simulink model "inv_im_param"  (R2026b)
settings: Solver=ode23tb  StopTime=param.sim.simlength  FixedStep=tc  MaxStep=param.glb_time.tc
values from neighbouring files (symbols this model uses):
  param = add_template_extras(param, options)    [init_model.m]
undefined symbols (not defined in the file or in its folder): magnitude
libraries: fl_lib x30, nesl_utility x13, lithium_ion_battery x1, induction_machine x1, dclink_with_center_tap x1, dead_time_generator_cmos_simulink x1, three_phase_pwm_modulator x1, three_phase_inverter_ideal_switch_based_model x1, three_phase_inverter_igbt_advanced_thermal_model x1, three_phase_inverter_mosfet_based_with_thermal_model x1, threephase_inductor_lib x1, simple_flexible_shaft x1
(part 1 of 3)
settings Model: Creator=dbagn  LastModifiedBy=d.bagnara
settings SolverCC: SolverResetMethod=Robust  ZeroCrossControl=DisableAll
settings DataIOCC: DSMLogging=off  ReturnWorkspaceOutputs=off  SaveOutput=off  SaveTime=off  SignalLogging=off
settings OptimizationCC: ReuseModelBlockBuffer=off
settings SFSimCC: CustomCodeUndefinedFunction=ThrowError  DefaultCustomCodeDeterministicFunctions=All
settings SFSimCC: SimCustomHeaderCode=|
  | #include "rpi.h"
  | #include "mavgflt.h"
  | #include "mavgflt_simulink.h"
  | #include "mavgflts.h"
  | #include "mavgflts_simulink.h"
  | #include "dsmavgflt.h"
  | #include "dsmavgflt_simulink.h"
  | #include "bemf_obsv.h"
  | #include "bemf_obsv_simulink.h"
  | #include "bemf_obsv_load_est.h"
  | #include "bemf_obsv_load_est_simulink.h"
  | #include "dqvector_pi.h"
  | #include "dqvector_pi_simulink.h"
  | #include "sv_pwm_simulink.h"
  | #include "sv_pwm.h"
  | #include "first_harmonic_tracker.h"
  | #include "first_harmonic_tracker_simulink.h"
  | #include "dqpll_thyr.h"
  | #include "dqpll_thyr_simulink.h"
  | #include "dqpll_grid.h"
  | #include "dqpll_grid_simulink.h"
settings SFSimCC: SimUserIncludeDirs=|
  | include
  | src
settings SFSimCC: SimUserSources=|
  | "rpi.c"
  | "mavgflt_simulink.c"
  | "mavgflt.c"
  | "mavgflts_simulink.c"
  | "mavgflts.c"
  | "dsmavgflt_simulink.c"
  | "dsmavgflt.c"
  | "bemf_obsv_simulink.c"
  | "bemf_obsv.c"
  | "bemf_obsv_load_est_simulink.c"
  | "bemf_obsv_load_est.c"
  | "dqvector_pi.c"
  | "dqvector_pi_simulink.c"
  | "sv_pwm_simulink.c"
  | "sv_pwm.c"
  | "first_harmonic_tracker_simulink.c"
  | "first_harmonic_tracker.c"
  | "dqpll_thyr_simulink.c"
  | "dqpll_thyr.c"
  | "dqpll_grid_simulink.c"
  | "dqpll_grid.c"
settings RTWCC: DLArmComputeVersion=19.05
settings SimscapeCC: SimscapeUseEnergyAccounting=off

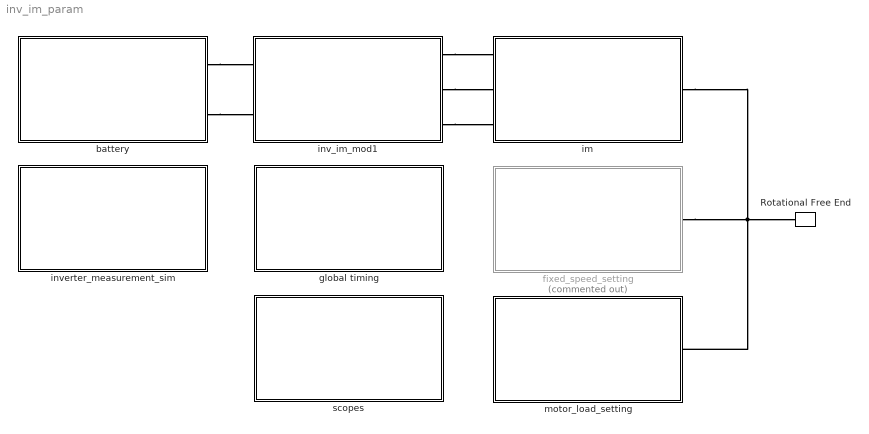
== system inv_im_param ==
  Rotational Free End : fl_lib/Mechanical/Rotational Elements/Rotational Free End  w_specify=off  w_priority=None  w=0 rad/s  w_nominal_specify=off  w_nominal_value=1  w_nominal_unit=rad/s
  battery : Subsystem
  fixed_speed_setting : Subsystem  Commented=on
  global timing : Subsystem
  im : Subsystem
  inv_im_mod1 : Subsystem
  inverter_measurement_sim : Subsystem
  motor_load_setting : Subsystem
  scopes : Subsystem
  connections:
  im/RConn1 -- motor_load_setting/LConn1 -- Rotational Free End/LConn1 -- fixed_speed_setting/LConn1
  inv_im_mod1/RConn2 -- im/LConn2
  inv_im_mod1/RConn1 -- im/LConn1
  inv_im_mod1/RConn3 -- im/LConn3
  battery/RConn1 -- inv_im_mod1/LConn1
  battery/RConn2 -- inv_im_mod1/LConn2

== system inv_im_param/battery ==
  Solver Configuration : nesl_utility/Solver Configuration  PhysicalDomain=network_engine_domain  SubClassName=solver  LeftPortType=input  RightPortType=generic  Tones=[]  Harmonics=[]  SimulateNoise=off  Profile=off  UseLocalSampling=off  EnableSwitchedLinearOptims=on  FrequencyDomain=off  UseCCode=off  RelTol=0.001  AbsTol=0.001  MinStep=1e-09  ToWorkspace=off  RevertToSquareIcSolve=off  NumHomotopyIterations=100  PhasorMode=off  PhasorModeNumHarmonics=1  ConsistencySolver=NEWTON_FTOL  CanonicalOrdering=UNORDERED  OptimizeIntermediates=UNOPTIMIZED  MulticoreSolverChoice=BACKWARD_EULER  IndexReductionMethod=DerivativeReplacement  DoDC=on  ResidualTolerance=1e-3  ConsistencyTolSource=GLOBAL  ConsistencyAbsTol=0.001  ConsistencyRelTol=0.001  ConsistencyTolFactor=0.001  UseLocalSolver=on  LocalSolverChoice=NE_BACKWARD_EULER_ADVANCER  ResolveIndetEquations=on  FunctionEvalNumThread=1  LocalSolverSampleTime=param.glb_time.tc  DoFixedCost=on  MaxNonlinIter=param.sim.nonlinear_iterations  MaxModeIter=2  ComputeImpulses=off  ImpulseIterations=2  LinearAlgebra=auto  LinearAlgebraNumThread=0  EquationFormulation=NE_TIME_EF  DelaysMemoryBudget=1024  AutomaticFiltering=on  FilteringTimeConstant=0.001  PartitionStorageMethod=AS_NEEDED  PartitionMemoryBudget=1024  PartitionMethod=BALANCED  MultibodyUseLocalSolver=off  MultibodyLocalSolverChoice=ODE1  MultibodyLocalSolverSampleTime=0.001
  To Workspace14 : ToWorkspace  VariableName=battery_data  SampleTime=param.glb_time.tc
      settings: MaxDataPoints=param.glb_time.Nc  Decimation=param.glb_time.decimation_tc
  lithium-ion_battery : lithium_ion_battery/lithium_ion_battery  Q=param.battery.pack_1.Q  number_of_cells=param.battery.pack_1.number_of_cells  E_1=param.battery.pack_1.E_1  E0=param.battery.pack_1.E0  E1=param.battery.pack_1.E1  E2=param.battery.pack_1.E2  E3=param.battery.pack_1.E3  Elog=param.battery.pack_1.Elog  R0=param.battery.pack_1.R0  R1=param.battery.pack_1.R1  C1=param.battery.pack_1.C1  M=param.battery.pack_1.M  alpha=param.battery.pack_1.alpha  soc_init=param.battery.pack_1.soc_init  ts_battery=param.glb_time.ts_dab  q1Kalman=param.battery.pack_1.q1Kalman  q2Kalman=param.battery.pack_1.q2Kalman  q3Kalman=param.battery.pack_1.q3Kalman  rKalman=param.battery.pack_1.rKalman  tc=param.glb_time.tc  enable_white_noise_m=0  battery_voltage_init_m=param.battery.nominal_battery_voltage_1
  litium ion battery : Scope
      settings: ActiveDisplayYMinimum=-388.27149612119968  ActiveDisplayYMaximum=1221.0011073633038  DataLoggingVariableName=ScopeData3
  single_phase_ui_measure : Subsystem
  dc+ : PMIOPort  Side=Right
  dc- : PMIOPort  Port=2  Side=Right
  wires:
  lithium-ion_battery/1 -> To Workspace14/1, litium ion battery/1
  connections:
  single_phase_ui_measure/LConn2 -- lithium-ion_battery/RConn2 -- Solver Configuration/RConn1
  single_phase_ui_measure/RConn1 -- dc+/RConn1
  lithium-ion_battery/RConn1 -- single_phase_ui_measure/LConn1
  dc-/RConn1 -- single_phase_ui_measure/RConn2

== system inv_im_param/fixed_speed_setting ==
  Ideal Angular Velocity Source : fl_lib/Mechanical/Mechanical Sources/Ideal Angular Velocity Source
  Mechanical Rotational Reference : fl_lib/Mechanical/Rotational Elements/Mechanical Rotational Reference
  PS Step1 : fl_lib/Physical Signals/Sources/PS Step  step_time=0.025 s  initial_value=0 rpm  final_value=param.load.rpm_sim rpm
  PS Transfer Function : fl_lib/Physical Signals/Linear Operators/PS Transfer Function  transfer_function_type=foundation.enum.transfer_function_type.lag  T=0.1 s  T1=2 s  T2=1 s  reset_method=foundation.enum.IntegratorResetSpec.None  initial_condition_spec=foundation.enum.IntegratorICSpec.Internal  y0=0 rpm
  shaft : PMIOPort  Side=Left
  connections:
  Mechanical Rotational Reference/LConn1 -- Ideal Angular Velocity Source/RConn2
  PS Step1/RConn1 -- PS Transfer Function/LConn1
  PS Transfer Function/RConn1 -- Ideal Angular Velocity Source/RConn1
  Ideal Angular Velocity Source/LConn1 -- shaft/RConn1

== system inv_im_param/global timing ==
  Unit Delay : UnitDelay  SampleTime=param.glb_time.tc
  Unit Delay1 : UnitDelay  SampleTime=param.glb_time.tc
  time_afe1 : Subsystem  mask{k=param.afe.behav.time_gain_module_1}
      mask prompts: k "Time Gain"
      mask Display:
      | disp('time-gen');
      | port_label('input', 1, 'crt');
      | port_label('output', 1, 'tout');
  time_afe3 : Subsystem  mask{k=1}
      mask prompts: k "Time Gain"
      mask Display:
      | disp('time-gen');
      | port_label('output', 1, 'tout');
  time_inv1 : Subsystem  mask{k=param.inv.behav.time_gain_module_2}
      mask prompts: k "Time Gain"
      mask Display:
      | disp('time-gen');
      | port_label('input', 1, 'crt');
      | port_label('output', 1, 'tout');
  tag scope: time_afe_module_1=global, time_inv_module_1=global, time_master=global
  wires:
  time_afe1/1(Out1) -> [time_afe_module_1]
  time_inv1/1(Out1) -> [time_inv_module_1]
  time_afe3/1(Out1) -> [time_master]
  [local_time_corr_afe1] -> Unit Delay/1
  Unit Delay/1 -> time_afe1/1(correction_time)
  [local_time_corr_inv1] -> Unit Delay1/1
  Unit Delay1/1 -> time_inv1/1(correction_time)

== system inv_im_param/im ==
  Bus Selector1 : BusSelector  OutputSignals=rotor_speed_electrical(rad/s)
  im_machine : Subsystem
  u : PMIOPort  Side=Left
  v : PMIOPort  Port=2  Side=Left
  w : PMIOPort  Port=3  Side=Left
  shaft : PMIOPort  Port=4  Side=Right
  tag scope: rotor_speed_electrical_im=global
  wires:
  im_machine/1(motor_data) -> Bus Selector1/1
  Bus Selector1/1 -> [rotor_speed_electrical_im]  "<rotor_speed_electrical(rad/s)>"
  connections:
  im_machine/LConn1 -- u/RConn1
  im_machine/LConn3 -- w/RConn1
  im_machine/LConn2 -- v/RConn1
  shaft/RConn1 -- im_machine/RConn1

== system inv_im_param/inv_im_mod1 ==
  dc_source : Subsystem
  inverter : Subsystem
  inverter_ctrl : Subsystem
  output_filter : Subsystem
  us_u : PMIOPort  Side=Right
  us_v : PMIOPort  Port=2  Side=Right
  us_w : PMIOPort  Port=3  Side=Right
  udc(+) : PMIOPort  Port=4  Side=Left
  udc(-) : PMIOPort  Port=5  Side=Left
  wires:
  inverter_ctrl/1(duvw_out) -> inverter/1(duvw)
  connections:
  inverter/LConn2 -- output_filter/RConn2
  inverter/LConn1 -- output_filter/RConn1
  inverter/LConn3 -- output_filter/RConn3
  output_filter/LConn2 -- us_v/RConn1
  output_filter/LConn3 -- us_w/RConn1
  output_filter/LConn1 -- us_u/RConn1
  dc_source/RConn1 -- inverter/RConn1
  inverter/RConn2 -- dc_source/RConn2
  dc_source/LConn2 -- udc(-)/RConn1
  dc_source/LConn1 -- udc(+)/RConn1

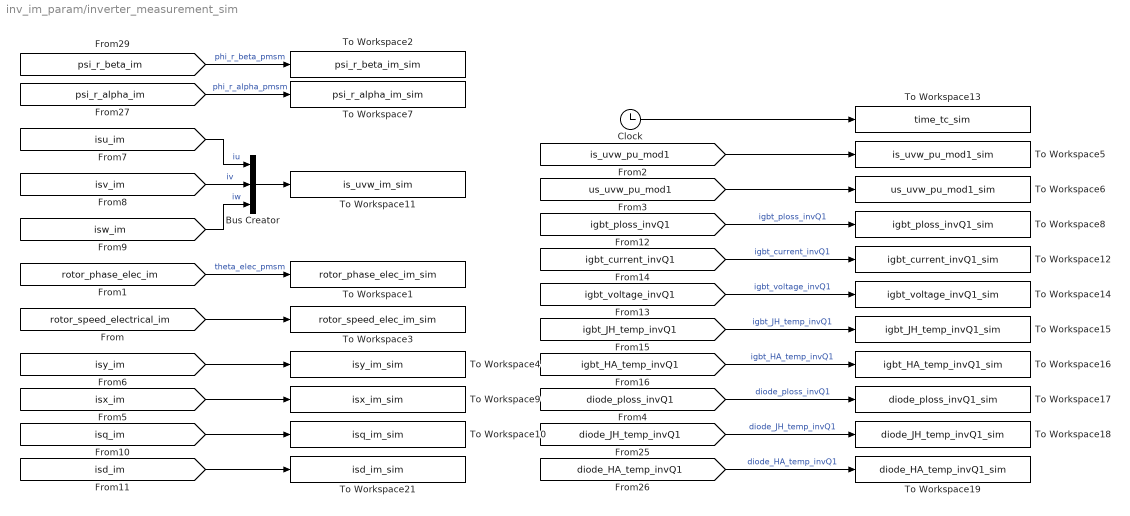
== system inv_im_param/inverter_measurement_sim ==
  Bus Creator : BusCreator  Inputs=3
  Clock : Clock
  To Workspace1 : ToWorkspace  VariableName=rotor_phase_elec_im_sim  SampleTime=param.glb_time.tc
      settings: MaxDataPoints=param.glb_time.Nc  Decimation=param.glb_time.decimation_tc
  To Workspace10 : ToWorkspace  VariableName=isq_im_sim  SampleTime=param.glb_time.tc
      settings: MaxDataPoints=param.glb_time.Nc  Decimation=param.glb_time.decimation_tc
  To Workspace11 : ToWorkspace  VariableName=is_uvw_im_sim  SampleTime=param.glb_time.tc
      settings: MaxDataPoints=param.glb_time.Nc  Decimation=param.glb_time.decimation_tc
  To Workspace12 : ToWorkspace  VariableName=igbt_current_invQ1_sim  SampleTime=param.glb_time.tc
      settings: MaxDataPoints=param.glb_time.Nc  Decimation=param.glb_time.decimation_tc
  To Workspace13 : ToWorkspace  VariableName=time_tc_sim  SampleTime=param.glb_time.tc
      settings: MaxDataPoints=param.glb_time.Nc  Decimation=param.glb_time.decimation_tc
  To Workspace14 : ToWorkspace  VariableName=igbt_voltage_invQ1_sim  SampleTime=param.glb_time.tc
      settings: MaxDataPoints=param.glb_time.Nc  Decimation=param.glb_time.decimation_tc
  To Workspace15 : ToWorkspace  VariableName=igbt_JH_temp_invQ1_sim  SampleTime=param.glb_time.tc
      settings: MaxDataPoints=param.glb_time.Nc  Decimation=param.glb_time.decimation_tc
  To Workspace16 : ToWorkspace  VariableName=igbt_HA_temp_invQ1_sim  SampleTime=param.glb_time.tc
      settings: MaxDataPoints=param.glb_time.Nc  Decimation=param.glb_time.decimation_tc
  To Workspace17 : ToWorkspace  VariableName=diode_ploss_invQ1_sim  SampleTime=param.glb_time.tc
      settings: MaxDataPoints=param.glb_time.Nc  Decimation=param.glb_time.decimation_tc
  To Workspace18 : ToWorkspace  VariableName=diode_JH_temp_invQ1_sim  SampleTime=param.glb_time.tc
      settings: MaxDataPoints=param.glb_time.Nc  Decimation=param.glb_time.decimation_tc
  To Workspace19 : ToWorkspace  VariableName=diode_HA_temp_invQ1_sim  SampleTime=param.glb_time.tc
      settings: MaxDataPoints=param.glb_time.Nc  Decimation=param.glb_time.decimation_tc
  To Workspace2 : ToWorkspace  VariableName=psi_r_beta_im_sim  SampleTime=param.glb_time.tc
      settings: MaxDataPoints=param.glb_time.Nc  Decimation=param.glb_time.decimation_tc
  To Workspace21 : ToWorkspace  VariableName=isd_im_sim  SampleTime=param.glb_time.tc
      settings: MaxDataPoints=param.glb_time.Nc  Decimation=param.glb_time.decimation_tc
  To Workspace3 : ToWorkspace  VariableName=rotor_speed_elec_im_sim  SampleTime=param.glb_time.tc
      settings: MaxDataPoints=param.glb_time.Nc  Decimation=param.glb_time.decimation_tc
  To Workspace4 : ToWorkspace  VariableName=isy_im_sim  SampleTime=param.glb_time.tc
      settings: MaxDataPoints=param.glb_time.Nc  Decimation=param.glb_time.decimation_tc
  To Workspace5 : ToWorkspace  VariableName=is_uvw_pu_mod1_sim  SampleTime=param.glb_time.tc
      settings: MaxDataPoints=param.glb_time.Nc  Decimation=param.glb_time.decimation_tc
  To Workspace6 : ToWorkspace  VariableName=us_uvw_pu_mod1_sim  SampleTime=param.glb_time.tc
      settings: MaxDataPoints=param.glb_time.Nc  Decimation=param.glb_time.decimation_tc
  To Workspace7 : ToWorkspace  VariableName=psi_r_alpha_im_sim  SampleTime=param.glb_time.tc
      settings: MaxDataPoints=param.glb_time.Nc  Decimation=param.glb_time.decimation_tc
  To Workspace8 : ToWorkspace  VariableName=igbt_ploss_invQ1_sim  SampleTime=param.glb_time.tc
      settings: MaxDataPoints=param.glb_time.Nc  Decimation=param.glb_time.decimation_tc
  To Workspace9 : ToWorkspace  VariableName=isx_im_sim  SampleTime=param.glb_time.tc
      settings: MaxDataPoints=param.glb_time.Nc  Decimation=param.glb_time.decimation_tc
  wires:
  [psi_r_alpha_im] -> To Workspace7/1  "phi_r_alpha_pmsm"
  [psi_r_beta_im] -> To Workspace2/1  "phi_r_beta_pmsm"
  [rotor_speed_electrical_im] -> To Workspace3/1
  [isv_im] -> Bus Creator/2  "iv"
  [isw_im] -> Bus Creator/3  "iw"
  [isu_im] -> Bus Creator/1  "iu"
  Bus Creator/1 -> To Workspace11/1
  [rotor_phase_elec_im] -> To Workspace1/1  "theta_elec_pmsm"
  [isy_im] -> To Workspace4/1
  [is_uvw_pu_mod1] -> To Workspace5/1
  [us_uvw_pu_mod1] -> To Workspace6/1
  [igbt_ploss_invQ1] -> To Workspace8/1  "igbt_ploss_invQ1"
  [igbt_current_invQ1] -> To Workspace12/1  "igbt_current_invQ1"
  [igbt_voltage_invQ1] -> To Workspace14/1  "igbt_voltage_invQ1"
  [igbt_JH_temp_invQ1] -> To Workspace15/1  "igbt_JH_temp_invQ1"
  [igbt_HA_temp_invQ1] -> To Workspace16/1  "igbt_HA_temp_invQ1"
  Clock/1 -> To Workspace13/1
  [diode_ploss_invQ1] -> To Workspace17/1  "diode_ploss_invQ1"
  [diode_JH_temp_invQ1] -> To Workspace18/1  "diode_JH_temp_invQ1"
  [diode_HA_temp_invQ1] -> To Workspace19/1  "diode_HA_temp_invQ1"
  [isx_im] -> To Workspace9/1
  [isq_im] -> To Workspace10/1
  [isd_im] -> To Workspace21/1

== system inv_im_param/motor_load_setting ==
  Gain : Gain  Gain=param.im.machine.pp
  Ideal Rotational Motion Sensor : fl_lib/Mechanical/Mechanical Sensors/Ideal Rotational Motion Sensor  reference=foundation.enum.MeasurementReference.difference  acceleration_port=false  velocity_port=true  position_port=true  wrap_angle=false  offset=0 rad
  Ideal Torque Source : fl_lib/Mechanical/Mechanical Sources/Ideal Torque Source
  Inertia : fl_lib/Mechanical/Rotational Elements/Inertia  inertia=param.load.external_load_inertia kg*m^2  num_ports=foundation.enum.numPorts2.one  w_specify=off  w_priority=High  w=0 rad/s  w_nominal_specify=off  w_nominal_value=1  w_nominal_unit=rad/s  t_specify=off  t_priority=None  t=0 N*m  t_nominal_specify=off  t_nominal_value=1  t_nominal_unit=N*m
  Integrator : Integrator
  Mechanical Rotational Reference : fl_lib/Mechanical/Rotational Elements/Mechanical Rotational Reference
  Mechanical Rotational Reference1 : fl_lib/Mechanical/Rotational Elements/Mechanical Rotational Reference
  PS Step : fl_lib/Physical Signals/Sources/PS Step  step_time=param.sim.load_step_time s  initial_value=1 N*m  final_value=1 N*m
  PS Transfer Function : fl_lib/Physical Signals/Linear Operators/PS Transfer Function  transfer_function_type=foundation.enum.transfer_function_type.lag  T=1 s  T1=2 s  T2=1 s  reset_method=foundation.enum.IntegratorResetSpec.None  initial_condition_spec=foundation.enum.IntegratorICSpec.Internal  y0=0 N*m
  PS-Simulink Converter : nesl_utility/PS-Simulink Converter  PhysicalDomain=network_engine_domain  SubClassName=ps_output  LeftPortType=input  RightPortType=output  PseudoPeriodic=off  Frequencies=[]  VectorFormat=1-D array  Unit=rad/s  AffineConversion=off
  PS-Simulink Converter1 : nesl_utility/PS-Simulink Converter  PhysicalDomain=network_engine_domain  SubClassName=ps_output  LeftPortType=input  RightPortType=output  PseudoPeriodic=off  Frequencies=[]  VectorFormat=1-D array  Unit=rpm  AffineConversion=off
  bounder1 : MATLAB Function  TreatAsAtomicUnit=on
  flexible_shaft : simple_flexible_shaft/flexible_shaft  b1=1  b2=1  J1=1  J2=1  b_displacement=1  k_displacement=1e5
  shaft : PMIOPort  Side=Left
  tag scope: encoder_electrical_phase=global, encoder_mechanical_speed=global
  wires:
  PS-Simulink Converter/1 -> Integrator/1
  Integrator/1 -> Gain/1
  Gain/1 -> bounder1/1(u)
  bounder1/1(y) -> [encoder_electrical_phase]
  PS-Simulink Converter1/1 -> [encoder_mechanical_speed]
  connections:
  Ideal Torque Source/LConn1 -- flexible_shaft/RConn1 -- Inertia/LConn1
  Ideal Torque Source/RConn2 -- Mechanical Rotational Reference/LConn1
  PS Transfer Function/RConn1 -- Ideal Torque Source/RConn1
  PS Step/RConn1 -- PS Transfer Function/LConn1
  flexible_shaft/LConn1 -- Ideal Rotational Motion Sensor/LConn1 -- shaft/RConn1
  Ideal Rotational Motion Sensor/RConn1 -- Mechanical Rotational Reference1/LConn1
  Ideal Rotational Motion Sensor/RConn2 -- PS-Simulink Converter1/LConn1 -- PS-Simulink Converter/LConn1

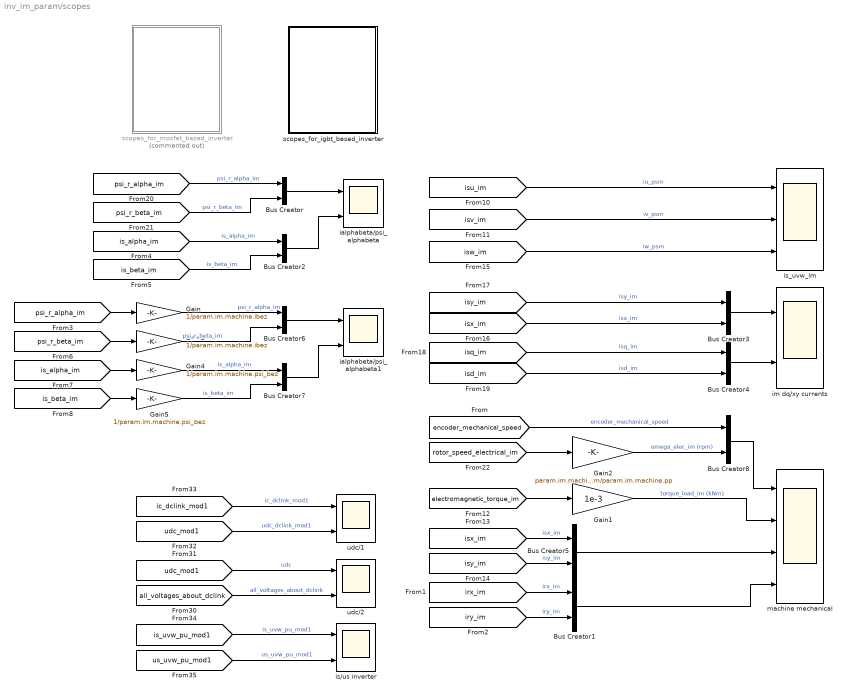
== system inv_im_param/scopes ==
  Bus Creator{,1..8} (9 alike) : BusCreator  Inputs=2
  Gain : Gain  Gain=1/param.im.machine.ibez
  Gain1 : Gain  Gain=1e-3
  Gain2 : Gain  Gain=param.im.machine.radpersecond2rpm/param.im.machine.pp
  Gain3 : Gain  Gain=1/param.im.machine.ibez
  Gain4 : Gain  Gain=1/param.im.machine.psi_bez
  Gain5 : Gain  Gain=1/param.im.machine.psi_bez
  ialphabeta/psi_alphabeta : Scope  NumInputPorts=2
      settings: SampleTime=param.glb_time.tc  ActiveDisplayYMinimum=-1.0786375199515998  ActiveDisplayYMaximum=1.0792953062694595  DataLoggingVariableName=ScopeData17
  ialphabeta/psi_alphabeta1 : Scope  NumInputPorts=2
      settings: SampleTime=param.glb_time.tc  ActiveDisplayYMinimum=-0.0018950393058757126  ActiveDisplayYMaximum=0.0018950920695159389  DataLoggingVariableName=ScopeData18
  im dq/xy currents : Scope  NumInputPorts=2
      settings: SampleTime=param.glb_time.tc  ActiveDisplayYMinimum=-1124.598311193791  ActiveDisplayYMaximum=1120.8872426827804  DataLoggingVariableName=ScopeData7
  is/us inverter : Scope  NumInputPorts=2
      settings: SampleTime=param.glb_time.tc  ActiveDisplayYMinimum=-1.8432109473411751  ActiveDisplayYMaximum=1.8312065303529172  DataLoggingVariableName=ScopeData11
  is_uvw_im : Scope  NumInputPorts=3
      settings: SampleTime=param.glb_time.tc  ActiveDisplayYMinimum=-1113.2920195668116  ActiveDisplayYMaximum=1113.31346416063  DataLoggingVariableName=ScopeData5
  machine mechanical : Scope  NumInputPorts=4
      settings: SampleTime=param.glb_time.tc  ActiveDisplayYMinimum=-18.632200322247279  ActiveDisplayYMaximum=2.78192242658902  DataLoggingVariableName=ScopeData6
  scopes_for_igbt_based_inverter : Subsystem
  scopes_for_mosfet_based_inverter : Subsystem  Commented=on
  udc/1 : Scope  NumInputPorts=2
      settings: SampleTime=param.glb_time.tc  ActiveDisplayYMinimum=-3641.314854214902  ActiveDisplayYMaximum=-3631.7131714883158  DataLoggingVariableName=ScopeData8
  udc/2 : Scope  NumInputPorts=2
      settings: SampleTime=param.glb_time.tc  ActiveDisplayYMinimum=628.98606143046629  ActiveDisplayYMaximum=672.06971446845785  DataLoggingVariableName=ScopeData9
  wires:
  [electromagnetic_torque_im] -> Gain1/1
  Bus Creator4/1 -> im dq/xy currents/2
  [isx_im] -> Bus Creator5/1  "isx_im"
  [isy_im] -> Bus Creator5/2  "isy_im"
  [isw_im] -> is_uvw_im/3  "iw_psm"
  [isd_im] -> Bus Creator4/2  "isd_im"
  [isv_im] -> is_uvw_im/2  "iv_psm"
  Bus Creator3/1 -> im dq/xy currents/1
  [isx_im] -> Bus Creator3/2  "isx_im"
  [isu_im] -> is_uvw_im/1  "iu_psm"
  [isy_im] -> Bus Creator3/1  "isy_im"
  [isq_im] -> Bus Creator4/1  "isq_im"
  [rotor_speed_electrical_im] -> Gain2/1
  [udc_mod1] -> udc/2/1  "udc"
  [ic_dclink_mod1] -> udc/1/1  "ic_dclink_mod1"
  [udc_mod1] -> udc/1/2  "udc_dclink_mod1"
  [all_voltages_about_dclink] -> udc/2/2  "all_voltages_about_dclink"
  [is_uvw_pu_mod1] -> is/us inverter/1  "is_uvw_pu_mod1"
  [us_uvw_pu_mod1] -> is/us inverter/2  "us_uvw_pu_mod1"
  [iry_im] -> Bus Creator1/2  "iry_im"
  [irx_im] -> Bus Creator1/1  "irx_im"
  [psi_r_alpha_im] -> Bus Creator/1  "psi_r_alpha_im"
  [psi_r_beta_im] -> Bus Creator/2  "psi_r_beta_im"
  [is_alpha_im] -> Bus Creator2/1  "is_alpha_im"
  [is_beta_im] -> Bus Creator2/2  "is_beta_im"
  Bus Creator/1 -> ialphabeta/psi_alphabeta/1
  Bus Creator2/1 -> ialphabeta/psi_alphabeta/2
  Bus Creator7/1 -> ialphabeta/psi_alphabeta1/2
  Bus Creator6/1 -> ialphabeta/psi_alphabeta1/1
  [is_beta_im] -> Gain5/1
  [is_alpha_im] -> Gain4/1
  [psi_r_beta_im] -> Gain3/1
  [psi_r_alpha_im] -> Gain/1
  Gain/1 -> Bus Creator6/1  "psi_r_alpha_im"
  Gain3/1 -> Bus Creator6/2  "psi_r_beta_im"
  Gain4/1 -> Bus Creator7/1  "is_alpha_im"
  Gain5/1 -> Bus Creator7/2  "is_beta_im"
  Gain2/1 -> Bus Creator8/2  "omega_elec_im (rpm)"
  [encoder_mechanical_speed] -> Bus Creator8/1  "encoder_mechanical_speed"
  Bus Creator8/1 -> machine mechanical/1
  Gain1/1 -> machine mechanical/2  "torque_load_im (kNm)"
  Bus Creator5/1 -> machine mechanical/3
  Bus Creator1/1 -> machine mechanical/4

== system inv_im_param/battery/single_phase_ui_measure ==
  Bus Creator : BusCreator  Inputs=2
  Current Sensor : fl_lib/Electrical/Electrical Sensors/Current Sensor
  Selector : Selector  InputPortWidth=2  IndexOptions=Index vector (dialog)  Indices=2  OutputSizes=1  RuntimeRangeChecks=off
  Selector1 : Selector  InputPortWidth=2  IndexOptions=Index vector (dialog)  Indices=1  OutputSizes=1  RuntimeRangeChecks=off
  Voltage Sensor : fl_lib/Electrical/Electrical Sensors/Voltage Sensor
  dab input modA : Scope  NumInputPorts=2
      settings: SampleTime=param.glb_time.tc  ActiveDisplayYMinimum=-413.54291450338707  ActiveDisplayYMaximum=396.93489435257015  DataLoggingVariableName=ScopeData2
  iph : nesl_utility/PS-Simulink Converter  PhysicalDomain=network_engine_domain  SubClassName=ps_output  LeftPortType=input  RightPortType=output  PseudoPeriodic=off  Frequencies=[]  VectorFormat=1-D array  Unit=A  AffineConversion=off
  uph : nesl_utility/PS-Simulink Converter  PhysicalDomain=network_engine_domain  SubClassName=ps_output  LeftPortType=input  RightPortType=output  PseudoPeriodic=off  Frequencies=[]  VectorFormat=1-D array  Unit=V  AffineConversion=off
  Udc(+) : PMIOPort  Side=Left
  udc(+) : PMIOPort  Port=2  Side=Right
  Udc(-) : PMIOPort  Port=3  Side=Left
  udc(-) : PMIOPort  Port=4  Side=Right
  tag scope: current_battery=global, voltage_battery=global
  wires:
  Bus Creator/1 -> Selector/1, Selector1/1  "ui_data"
  iph/1 -> Bus Creator/1  "iph"
  uph/1 -> Bus Creator/2  "uph"
  Selector1/1 -> [current_battery], dab input modA/1  "current_battery"
  Selector/1 -> dab input modA/2, [voltage_battery]  "voltage_battery"
  connections:
  iph/LConn1 -- Current Sensor/RConn1
  Voltage Sensor/LConn1 -- Current Sensor/LConn1 -- Udc(+)/RConn1
  Current Sensor/RConn2 -- udc(+)/RConn1
  Voltage Sensor/RConn1 -- uph/LConn1
  Voltage Sensor/RConn2 -- Udc(-)/RConn1 -- udc(-)/RConn1

== system inv_im_param/global timing/time_afe1 ==
  correction_time : Inport
  Constant : Constant
  Gain : Gain  Gain=k
  Product : Product
  Sum : Sum  Inputs=|++
  time_1 : Clock
  Out1 : Outport
  wires:
  time_1/1 -> Gain/1
  Gain/1 -> Product/1
  Product/1 -> Out1/1
  correction_time/1 -> Sum/1
  Sum/1 -> Product/2
  Constant/1 -> Sum/2

== system inv_im_param/global timing/time_afe3 ==
  Gain : Gain  Gain=k
  time_1 : Clock
  Out1 : Outport
  wires:
  Gain/1 -> Out1/1
  time_1/1 -> Gain/1

== system inv_im_param/global timing/time_inv1 ==
  correction_time : Inport
  Constant : Constant
  Gain : Gain  Gain=k
  Product : Product
  Sum : Sum  Inputs=|++
  time_1 : Clock
  Out1 : Outport
  wires:
  time_1/1 -> Gain/1
  Gain/1 -> Product/1
  Product/1 -> Out1/1
  correction_time/1 -> Sum/1
  Constant/1 -> Sum/2
  Sum/1 -> Product/2

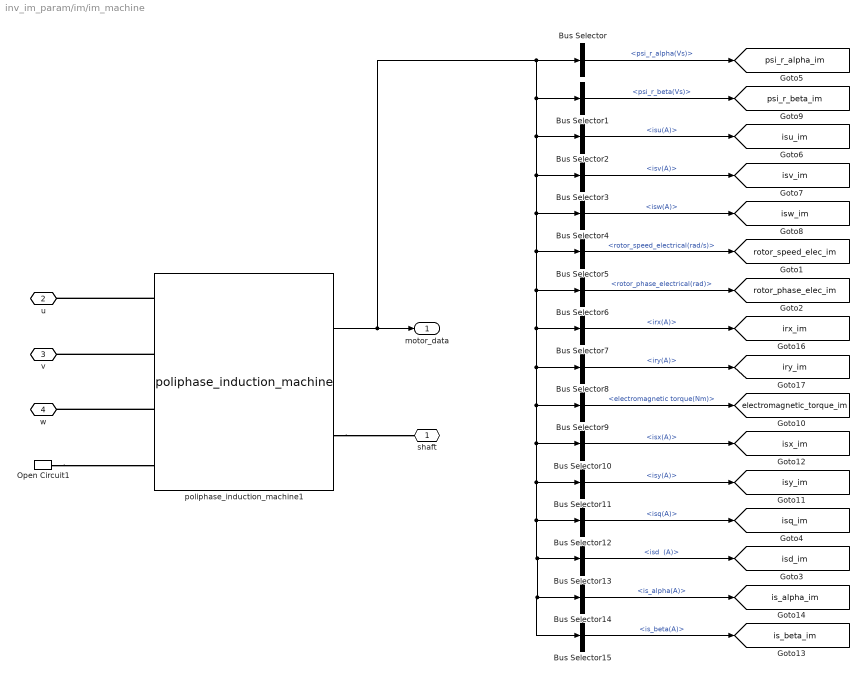
== system inv_im_param/im/im_machine ==
  Bus Selector : BusSelector  OutputSignals=psi_r_alpha(Vs)
  Bus Selector1 : BusSelector  OutputSignals=psi_r_beta(Vs)
  Bus Selector10 : BusSelector  OutputSignals=isx(A)
  Bus Selector11 : BusSelector  OutputSignals=isy(A)
  Bus Selector12 : BusSelector  OutputSignals=isq(A)
  Bus Selector13 : BusSelector  OutputSignals="isd  (A)"
  Bus Selector14 : BusSelector  OutputSignals=is_alpha(A)
  Bus Selector15 : BusSelector  OutputSignals=is_beta(A)
  Bus Selector2 : BusSelector  OutputSignals=isu(A)
  Bus Selector3 : BusSelector  OutputSignals=isv(A)
  Bus Selector4 : BusSelector  OutputSignals=isw(A)
  Bus Selector5 : BusSelector  OutputSignals=rotor_speed_electrical(rad/s)
  Bus Selector6 : BusSelector  OutputSignals=rotor_phase_electrical(rad)
  Bus Selector7 : BusSelector  OutputSignals=irx(A)
  Bus Selector8 : BusSelector  OutputSignals=iry(A)
  Bus Selector9 : BusSelector  OutputSignals=electromagnetic torque(Nm)
  Open Circuit1 : fl_lib/Electrical/Electrical Elements/Open Circuit  v_specify=off  v_priority=None  v=0 V  v_nominal_specify=off  v_nominal_value=1  v_nominal_unit=V
  poliphase_induction_machine1 : induction_machine/poliphase_induction_machine  Rs_m=param.im.machine.Rs  Ls_m=param.im.machine.Ls  Lm_m=param.im.machine.Lm  Lr_m=param.im.machine.Lr  Rr_m=param.im.machine.Rr  Jm_m=param.im.machine.Jm  bm_m=param.im.machine.load_friction  cp_m=param.im.machine.pp
  shaft : PMIOPort  Side=Right
  u : PMIOPort  Port=2  Side=Left
  v : PMIOPort  Port=3  Side=Left
  w : PMIOPort  Port=4  Side=Left
  motor_data : Outport
  tag scope: electromagnetic_torque_im=global, irx_im=global, iry_im=global, is_alpha_im=global, is_beta_im=global, isd_im=global, isq_im=global, isu_im=global, isv_im=global, isw_im=global, isx_im=global, isy_im=global, psi_r_alpha_im=global, psi_r_beta_im=global, rotor_phase_elec_im=global, rotor_speed_elec_im=global
  wires:
  Bus Selector/1 -> [psi_r_alpha_im]  "<psi_r_alpha(Vs)>"
  Bus Selector1/1 -> [psi_r_beta_im]  "<psi_r_beta(Vs)>"
  Bus Selector2/1 -> [isu_im]  "<isu(A)>"
  Bus Selector3/1 -> [isv_im]  "<isv(A)>"
  Bus Selector4/1 -> [isw_im]  "<isw(A)>"
  Bus Selector5/1 -> [rotor_speed_elec_im]  "<rotor_speed_electrical(rad/s)>"
  Bus Selector6/1 -> [rotor_phase_elec_im]  "<rotor_phase_electrical(rad)>"
  Bus Selector9/1 -> [electromagnetic_torque_im]  "<electromagnetic torque(Nm)>"
  Bus Selector12/1 -> [isq_im]  "<isq(A)>"
  Bus Selector13/1 -> [isd_im]  "<isd  (A)>"
  Bus Selector10/1 -> [isx_im]  "<isx(A)>"
  Bus Selector11/1 -> [isy_im]  "<isy(A)>"
  Bus Selector7/1 -> [irx_im]  "<irx(A)>"
  Bus Selector8/1 -> [iry_im]  "<iry(A)>"
  Bus Selector15/1 -> [is_beta_im]  "<is_beta(A)>"
  Bus Selector14/1 -> [is_alpha_im]  "<is_alpha(A)>"
  poliphase_induction_machine1/1 -> Bus Selector8/1, Bus Selector10/1, Bus Selector11/1, Bus Selector12/1, Bus Selector15/1, Bus Selector14/1, Bus Selector13/1, Bus Selector9/1, Bus Selector7/1, Bus Selector6/1, Bus Selector5/1, Bus Selector4/1, Bus Selector3/1, Bus Selector2/1, Bus Selector1/1, Bus Selector/1, motor_data/1
  connections:
  poliphase_induction_machine1/RConn1 -- shaft/RConn1
  poliphase_induction_machine1/LConn1 -- u/RConn1
  poliphase_induction_machine1/LConn2 -- v/RConn1
  poliphase_induction_machine1/LConn3 -- w/RConn1
  Open Circuit1/LConn1 -- poliphase_induction_machine1/LConn4

== system inv_im_param/inv_im_mod1/dc_source ==
  Bus Selector : BusSelector  OutputSignals=udc,Cdc1_current,vdc_pu
  Electrical Reference : fl_lib/Electrical/Electrical Elements/Electrical Reference
  dclink : dclink_with_center_tap/dclink  Cdc1=param.afe.hw.CFi1  Cdc2=param.afe.hw.CFi2  Rudc_measure=107e3  Vdc_scale=param.afe.hw.udc_nom
  udc(+) : PMIOPort  Side=Right
  udc(-) : PMIOPort  Port=2  Side=Right
  Udc(+) : PMIOPort  Port=3  Side=Left
  Udc(-) : PMIOPort  Port=4  Side=Left
  tag scope: all_voltages_about_dclink=global, ic_dclink_mod1=global, udc_mod1=global, vdc_pu_inv_mod1=global
  wires:
  dclink/1 -> Bus Selector/1, [all_voltages_about_dclink]
  Bus Selector/1 -> [udc_mod1]  "<udc>"
  Bus Selector/2 -> [ic_dclink_mod1]  "<Cdc1_current>"
  Bus Selector/3 -> [vdc_pu_inv_mod1]  "<vdc_pu>"
  connections:
  dclink/LConn1 -- udc(+)/RConn1
  Electrical Reference/LConn1 -- dclink/RConn2
  udc(-)/RConn1 -- dclink/LConn2
  dclink/RConn3 -- Udc(-)/RConn1
  dclink/RConn1 -- Udc(+)/RConn1

== system inv_im_param/inv_im_mod1/inverter ==
  duvw : Inport
  Current Sensor : fl_lib/Electrical/Electrical Sensors/Current Sensor
  PS-Simulink Converter1 : nesl_utility/PS-Simulink Converter  PhysicalDomain=network_engine_domain  SubClassName=ps_output  LeftPortType=input  RightPortType=output  PseudoPeriodic=off  Frequencies=[]  VectorFormat=1-D array  Unit=A  AffineConversion=on
  PS-Simulink Converter4 : nesl_utility/PS-Simulink Converter  PhysicalDomain=network_engine_domain  SubClassName=ps_output  LeftPortType=input  RightPortType=output  PseudoPeriodic=off  Frequencies=[]  VectorFormat=1-D array  Unit=V  AffineConversion=on
  To Workspace : ToWorkspace  VariableName=idc_sim_mod1  SampleTime=param.glb_time.tc
      settings: MaxDataPoints=param.glb_time.Nc  Decimation=param.glb_time.decimation_tc
  To Workspace1 : ToWorkspace  VariableName=udc_sim_mod1  SampleTime=param.glb_time.tc
      settings: MaxDataPoints=param.glb_time.Nc  Decimation=param.glb_time.decimation_tc
  Transfer Fcn : TransferFcn  Denominator=[1e-2 1]
  Voltage Sensor : fl_lib/Electrical/Electrical Sensors/Voltage Sensor
  idc/udc : Scope  NumInputPorts=2
      settings: SampleTime=param.glb_time.tc  ActiveDisplayYMinimum=-35.93464770956853  ActiveDisplayYMaximum=323.41182938611684
  inverter : Subsystem
  Udc(+) : PMIOPort  Side=Right
  Udc(-) : PMIOPort  Port=2  Side=Right
  us_u : PMIOPort  Port=3  Side=Left
  us_v : PMIOPort  Port=4  Side=Left
  us_w : PMIOPort  Port=5  Side=Left
  wires:
  PS-Simulink Converter4/1 -> To Workspace1/1, idc/udc/2  "udc"
  PS-Simulink Converter1/1 -> Transfer Fcn/1  "idc"
  Transfer Fcn/1 -> To Workspace/1, idc/udc/1  "idc_flt"
  duvw/1 -> inverter/1(gate_cmds_uvw)
  connections:
  PS-Simulink Converter4/LConn1 -- Voltage Sensor/RConn1
  us_u/RConn1 -- inverter/LConn1
  us_v/RConn1 -- inverter/LConn2
  us_w/RConn1 -- inverter/LConn3
  Voltage Sensor/RConn2 -- inverter/RConn2 -- Udc(-)/RConn1
  Current Sensor/LConn1 -- Udc(+)/RConn1
  Voltage Sensor/LConn1 -- inverter/RConn1 -- Current Sensor/RConn2
  PS-Simulink Converter1/LConn1 -- Current Sensor/RConn1

== system inv_im_param/inv_im_mod1/inverter_ctrl ==
  im_control : Subsystem
  duvw_out : Outport
  tag scope: local_time_corr_inv1=global, master_torque_ref=global
  wires:
  [is_uvw_pu_mod1] -> im_control/1(is_uvw)
  [TRGO_inv_module_1] -> im_control/Trigger
  [vdc_pu_inv_mod1] -> im_control/2(udc_pu)
  im_control/1(duvw) -> duvw_out/1
  [time_inv_module_1] -> im_control/3(local_time)
  [time_master] -> im_control/4(master_time)
  im_control/2(local_time_corr) -> [local_time_corr_inv1]
  im_control/3(master_torque_ref) -> [master_torque_ref]
  [encoder_electrical_phase] -> im_control/5(rotor_phase_elec_im)
  [rotor_speed_elec_im] -> im_control/6(rotor_speed_elec_im)

== system inv_im_param/inv_im_mod1/output_filter ==
  Inductor{,1..5} (6 alike) : fl_lib/Electrical/Electrical Elements/Inductor  l=1e-6 H  r=0 Ohm  g=1e-9 1/Ohm  i_specify=off  i_priority=None  i=0 A  i_nominal_specify=off  i_nominal_value=1  i_nominal_unit=A  v_specify=off  v_priority=None  v=0 V  v_nominal_specify=off  v_nominal_value=1  v_nominal_unit=V  i_L_specify=off  i_L_priority=High  i_L=0 A  i_L_nominal_specify=off  i_L_nominal_value=1  i_L_nominal_unit=A
  threephase inductor : threephase_inductor_lib/threephase inductor  Lp=param.inv.hw.LFi H  L0=param.inv.hw.LFi_cm H  Rp=param.inv.hw.RLFi Ohm  R0=param.inv.hw.RLFi_cm Ohm  Lls=5e-6 H  uu_1_specify=off  uu_1_priority=None  uu_1=0 V  uu_1_nominal_specify=off  uu_1_nominal_value=1  uu_1_nominal_unit=V  uv_1_specify=off  uv_1_priority=None  uv_1=0 V  uv_1_nominal_specify=off  uv_1_nominal_value=1  uv_1_nominal_unit=V  uw_1_specify=off  uw_1_priority=None  uw_1=0 V  uw_1_nominal_specify=off  uw_1_nominal_value=1  uw_1_nominal_unit=V  uu_2_specify=off  uu_2_priority=None  uu_2=0 V  uu_2_nominal_specify=off  uu_2_nominal_value=1  uu_2_nominal_unit=V  uv_2_specify=off  uv_2_priority=None  uv_2=0 V  uv_2_nominal_specify=off  uv_2_nominal_value=1  uv_2_nominal_unit=V  uw_2_specify=off  uw_2_priority=None  uw_2=0 V  uw_2_nominal_specify=off  uw_2_nominal_value=1  uw_2_nominal_unit=V  iu_specify=off  iu_priority=None  iu=0 A  iu_nominal_specify=off  iu_nominal_value=1  iu_nominal_unit=A  iv_specify=off  iv_priority=None  iv=0 A  iv_nominal_specify=off  iv_nominal_value=1  iv_nominal_unit=A  iw_specify=off  iw_priority=None  iw=0 A  iw_nominal_specify=off  iw_nominal_value=1  iw_nominal_unit=A
  threephase_vi_measures_stack : Subsystem
  us_u : PMIOPort  Side=Left
  uu : PMIOPort  Port=2  Side=Right
  us_v : PMIOPort  Port=3  Side=Left
  uv : PMIOPort  Port=4  Side=Right
  us_w : PMIOPort  Port=5  Side=Left
  uw : PMIOPort  Port=6  Side=Right
  connections:
  threephase_vi_measures_stack/LConn1 -- us_u/RConn1
  threephase_vi_measures_stack/LConn2 -- us_v/RConn1
  threephase_vi_measures_stack/LConn3 -- us_w/RConn1
  Inductor3/LConn1 -- threephase_vi_measures_stack/RConn1
  threephase inductor/LConn2 -- Inductor4/RConn1
  threephase inductor/LConn3 -- Inductor5/RConn1
  threephase inductor/RConn1 -- Inductor/LConn1
  threephase inductor/RConn2 -- Inductor1/LConn1
  threephase inductor/RConn3 -- Inductor2/LConn1
  Inductor/RConn1 -- uu/RConn1
  Inductor1/RConn1 -- uv/RConn1
  Inductor2/RConn1 -- uw/RConn1
  threephase inductor/LConn1 -- Inductor3/RConn1
  Inductor4/LConn1 -- threephase_vi_measures_stack/RConn2
  Inductor5/LConn1 -- threephase_vi_measures_stack/RConn3

== system inv_im_param/scopes/scopes_for_igbt_based_inverter ==
  Bus Creator1 : BusCreator  Inputs=2
  Bus Creator2 : BusCreator  Inputs=2
  Bus Creator6 : BusCreator  Inputs=2
  diode power losses INV Q1 : Scope  NumInputPorts=2
      settings: SampleTime=param.glb_time.tc  ActiveDisplayYMinimum=-521.65205354232455  ActiveDisplayYMaximum=4694.8657991887039  DataLoggingVariableName=ScopeData4
  igbt power losses INV Q1 : Scope  NumInputPorts=4
      settings: SampleTime=param.glb_time.tc  ActiveDisplayYMinimum=-428.52278754268491  ActiveDisplayYMaximum=366.44991331174913  DataLoggingVariableName=ScopeData16
  igbt power losses INV Q2 : Scope  NumInputPorts=4
      settings: SampleTime=param.glb_time.tc  ActiveDisplayYMinimum=-187.00455358192744  ActiveDisplayYMaximum=1683.5427783442003
  wires:
  [diode_JH_temp_invQ1] -> Bus Creator6/1  "diode_JH_temp_invQ1"
  [diode_ploss_invQ1] -> diode power losses INV Q1/1  "diode_ploss_invQ1"
  Bus Creator2/1 -> igbt power losses INV Q1/4
  [diode_HA_temp_invQ1] -> Bus Creator6/2  "diode_HA_temp_invQ1"
  [igbt_current_invQ1] -> igbt power losses INV Q1/2  "igbt_current_invQ1"
  [igbt_HA_temp_invQ1] -> Bus Creator2/2  "igbt_HA_temp_invQ1"
  Bus Creator1/1 -> igbt power losses INV Q2/4
  [igbt_voltage_invQ1] -> igbt power losses INV Q1/3  "igbt_voltage_invQ1"
  [igbt_JH_temp_invQ2] -> Bus Creator1/1  "igbt_JH_temp_invQ2"
  [igbt_current_invQ2] -> igbt power losses INV Q2/2  "igbt_current_invQ2"
  [igbt_ploss_invQ1] -> igbt power losses INV Q1/1  "igbt_ploss_invQ1"
  [igbt_HA_temp_invQ2] -> Bus Creator1/2  "igbt_HA_temp_invQ2"
  [igbt_JH_temp_invQ1] -> Bus Creator2/1  "igbt_JH_temp_invQ1"
  [igbt_ploss_invQ2] -> igbt power losses INV Q2/1  "igbt_ploss_invQ2"
  [igbt_voltage_invQ2] -> igbt power losses INV Q2/3  "igbt_voltage_invQ2"
  Bus Creator6/1 -> diode power losses INV Q1/2

== system inv_im_param/scopes/scopes_for_mosfet_based_inverter ==
  Bus Creator8 : BusCreator  Inputs=2
  Bus Creator9 : BusCreator  Inputs=2
  mosfet power losses INV Q1 : Scope  NumInputPorts=4
      settings: SampleTime=param.glb_time.tc  ActiveDisplayYMinimum=-32.258190719935513  ActiveDisplayYMaximum=388.05311151106906  DataLoggingVariableName=ScopeData28
  mosfet power losses INV Q2 : Scope  NumInputPorts=4
      settings: SampleTime=param.glb_time.tc  ActiveDisplayYMinimum=-60.051099059926763  ActiveDisplayYMaximum=540.45256909803  DataLoggingVariableName=ScopeData29
  wires:
  [mosfet_JH_temp_invQ1] -> Bus Creator8/1  "mosfet_JH_temp_invQ1"
  Bus Creator9/1 -> mosfet power losses INV Q2/4
  [mosfet_HA_temp_invQ2] -> Bus Creator9/2  "mosfet_HA_temp_invQ2"
  [mosfet_HA_temp_invQ1] -> Bus Creator8/2  "mosfet_HA_temp_invQ1"
  [mosfet_ploss_invQ2] -> mosfet power losses INV Q2/1  "mosfet_ploss_invQ2"
  [mosfet_JH_temp_invQ2] -> Bus Creator9/1  "mosfet_JH_temp_invQ2"
  [mosfet_current_invQ2] -> mosfet power losses INV Q2/3  "mosfet_current_invQ2"
  [mosfet_ploss_invQ1] -> mosfet power losses INV Q1/1  "mosfet_ploss_invQ1"
  [mosfet_voltage_invQ2] -> mosfet power losses INV Q2/2  "mosfet_voltage_invQ2"
  [mosfet_current_invQ1] -> mosfet power losses INV Q1/3  "mosfet_current_invQ1"
  Bus Creator8/1 -> mosfet power losses INV Q1/4
  [mosfet_voltage_invQ1] -> mosfet power losses INV Q1/2  "mosfet_voltage_invQ1"

== system inv_im_param/inv_im_mod1/inverter/inverter ==
  gate_cmds_uvw : Inport
  dead_time_generator_cmos_simulink : dead_time_generator_cmos_simulink/dead_time_generator_cmos_simulink  Commented=through  ts=param.glb_time.tc  positive_voltage_rail=15  dead_time=param.glb_time.dead_time_INV
  sv_pwm : Subsystem
  three_phase_inverter_ideal_switch_based_model : three_phase_inverter_ideal_switch_based_model/three phase inverter ideal switch based model  Ron_ideal_switch=param.inv.ideal_switch.Rds_on  Vth=param.inv.ideal_switch.Vth  Vgamma=param.inv.ideal_switch.Vdon_diode  Rdon_diode=param.inv.ideal_switch.Rdon_diode  Csnubber=param.inv.ideal_switch.Csnubber  Rsnubber=param.inv.ideal_switch.Rsnubber
  three_phase_inverter_igbt_adv_thermal_model : Subsystem  Commented=on
  three_phase_inverter_mosfet_based_with_thermal_model : Subsystem  Commented=on
  u : PMIOPort  Side=Left
  v : PMIOPort  Port=2  Side=Left
  w : PMIOPort  Port=3  Side=Left
  udc(+) : PMIOPort  Port=4  Side=Right
  udc(-) : PMIOPort  Port=5  Side=Right
  wires:
  sv_pwm/1(gate_cmds) -> dead_time_generator_cmos_simulink/1
  gate_cmds_uvw/1 -> sv_pwm/1(gate_cmds_uvw)
  dead_time_generator_cmos_simulink/1 -> three_phase_inverter_mosfet_based_with_thermal_model/1(gate_commands), three_phase_inverter_igbt_adv_thermal_model/1(gate_commands), three_phase_inverter_ideal_switch_based_model/1
  connections:
  udc(+)/RConn1 -- three_phase_inverter_ideal_switch_based_model/LConn1 -- three_phase_inverter_igbt_adv_thermal_model/LConn1 -- three_phase_inverter_mosfet_based_with_thermal_model/LConn1
  udc(-)/RConn1 -- three_phase_inverter_ideal_switch_based_model/LConn2 -- three_phase_inverter_igbt_adv_thermal_model/LConn2 -- three_phase_inverter_mosfet_based_with_thermal_model/LConn2
  u/RConn1 -- three_phase_inverter_igbt_adv_thermal_model/RConn1 -- three_phase_inverter_mosfet_based_with_thermal_model/RConn1 -- three_phase_inverter_ideal_switch_based_model/RConn1
  v/RConn1 -- three_phase_inverter_igbt_adv_thermal_model/RConn2 -- three_phase_inverter_mosfet_based_with_thermal_model/RConn2 -- three_phase_inverter_ideal_switch_based_model/RConn2
  w/RConn1 -- three_phase_inverter_igbt_adv_thermal_model/RConn3 -- three_phase_inverter_ideal_switch_based_model/RConn3 -- three_phase_inverter_mosfet_based_with_thermal_model/RConn3

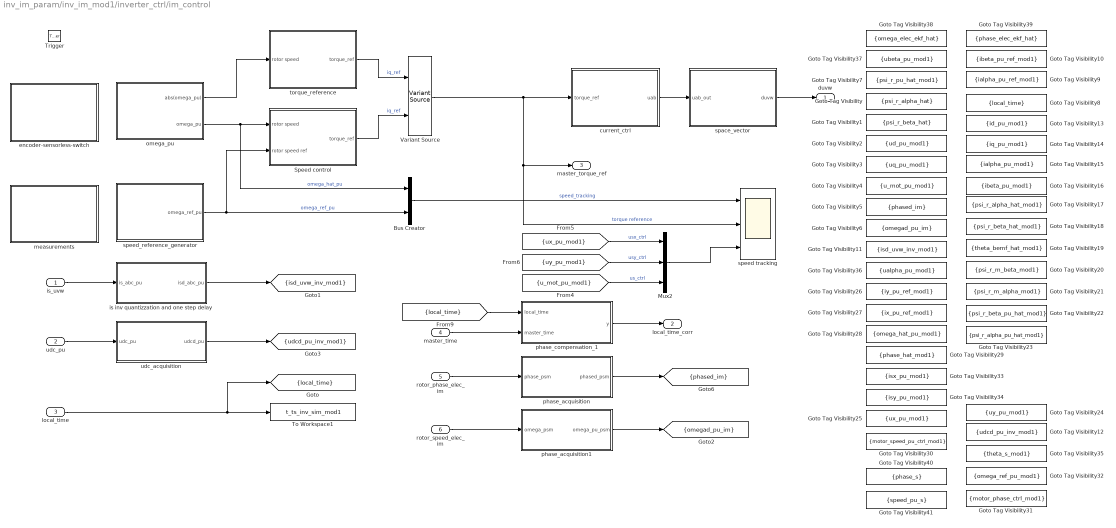
== system inv_im_param/inv_im_mod1/inverter_ctrl/im_control ==
  is_uvw : Inport
  udc_pu : Inport  Port=2
  local_time : Inport  Port=3
  master_time : Inport  Port=4
  rotor_phase_elec_im : Inport  Port=5
  rotor_speed_elec_im : Inport  Port=6
  Trigger : TriggerPort  VariantControl=(inherit)  PortDimensions=1
  Bus Creator : BusCreator  Inputs=2
  Goto Tag Visibility : GotoTagVisibility  GotoTag=psi_r_alpha_hat
  Goto Tag Visibility1 : GotoTagVisibility  GotoTag=psi_r_beta_hat
  Goto Tag Visibility10 : GotoTagVisibility  GotoTag=ibeta_pu_ref_mod1
  Goto Tag Visibility11 : GotoTagVisibility  GotoTag=isd_uvw_inv_mod1
  Goto Tag Visibility12 : GotoTagVisibility  GotoTag=udcd_pu_inv_mod1
  Goto Tag Visibility13 : GotoTagVisibility  GotoTag=id_pu_mod1
  Goto Tag Visibility14 : GotoTagVisibility  GotoTag=iq_pu_mod1
  Goto Tag Visibility15 : GotoTagVisibility  GotoTag=ialpha_pu_mod1
  Goto Tag Visibility16 : GotoTagVisibility  GotoTag=ibeta_pu_mod1
  Goto Tag Visibility17 : GotoTagVisibility  GotoTag=psi_r_alpha_hat_mod1
  Goto Tag Visibility18 : GotoTagVisibility  GotoTag=psi_r_beta_hat_mod1
  Goto Tag Visibility19 : GotoTagVisibility  GotoTag=theta_bemf_hat_mod1
  Goto Tag Visibility2 : GotoTagVisibility  GotoTag=ud_pu_mod1
  Goto Tag Visibility20 : GotoTagVisibility  GotoTag=psi_r_m_beta_mod1
  Goto Tag Visibility21 : GotoTagVisibility  GotoTag=psi_r_m_alpha_mod1
  Goto Tag Visibility22 : GotoTagVisibility  GotoTag=psi_r_beta_pu_hat_mod1
  Goto Tag Visibility23 : GotoTagVisibility  GotoTag=psi_r_alpha_pu_hat_mod1
  Goto Tag Visibility24 : GotoTagVisibility  GotoTag=uy_pu_mod1
  Goto Tag Visibility25 : GotoTagVisibility  GotoTag=ux_pu_mod1
  Goto Tag Visibility26 : GotoTagVisibility  GotoTag=iy_pu_ref_mod1
  Goto Tag Visibility27 : GotoTagVisibility  GotoTag=ix_pu_ref_mod1
  Goto Tag Visibility28 : GotoTagVisibility  GotoTag=omega_hat_pu_mod1
  Goto Tag Visibility29 : GotoTagVisibility  GotoTag=phase_hat_mod1
  Goto Tag Visibility3 : GotoTagVisibility  GotoTag=uq_pu_mod1
  Goto Tag Visibility30 : GotoTagVisibility  GotoTag=motor_speed_pu_ctrl_mod1
  Goto Tag Visibility31 : GotoTagVisibility  GotoTag=motor_phase_ctrl_mod1
  Goto Tag Visibility32 : GotoTagVisibility  GotoTag=omega_ref_pu_mod1
  Goto Tag Visibility33 : GotoTagVisibility  GotoTag=isx_pu_mod1
  Goto Tag Visibility34 : GotoTagVisibility  GotoTag=isy_pu_mod1
  Goto Tag Visibility35 : GotoTagVisibility  GotoTag=theta_s_mod1
  Goto Tag Visibility36 : GotoTagVisibility  GotoTag=ualpha_pu_mod1
  Goto Tag Visibility37 : GotoTagVisibility  GotoTag=ubeta_pu_mod1
  Goto Tag Visibility38 : GotoTagVisibility  GotoTag=omega_elec_ekf_hat
  Goto Tag Visibility39 : GotoTagVisibility  GotoTag=phase_elec_ekf_hat
  Goto Tag Visibility4 : GotoTagVisibility  GotoTag=u_mot_pu_mod1
  Goto Tag Visibility40 : GotoTagVisibility  GotoTag=phase_s
  Goto Tag Visibility41 : GotoTagVisibility  GotoTag=speed_pu_s
  Goto Tag Visibility5 : GotoTagVisibility  GotoTag=phased_im
  Goto Tag Visibility6 : GotoTagVisibility  GotoTag=omegad_pu_im
  Goto Tag Visibility7 : GotoTagVisibility  GotoTag=psi_r_pu_hat_mod1
  Goto Tag Visibility8 : GotoTagVisibility  GotoTag=local_time
  Goto Tag Visibility9 : GotoTagVisibility  GotoTag=ialpha_pu_ref_mod1
  Mux2 : Mux  Inputs=3
  Speed control : Subsystem
  To Workspace1 : ToWorkspace  VariableName=t_ts_inv_sim_mod1  SampleTime=-1
      settings: MaxDataPoints=param.glb_time.Ns_afe
  Variant Source : VariantSource  VariantControls={param.im.mode.use_torque_curve == 1, param.im.mode.use_speed_control == 1}
  current_ctrl : Subsystem
  encoder-sensorless-switch : Subsystem
  is inv quantizzation and one step delay : Subsystem
  measurements : Subsystem
  omega_pu : Subsystem
  phase_acquisition : Subsystem
  phase_acquisition1 : Subsystem
  phase_compensation_1 : Subsystem
  space_vector : Subsystem
  speed tracking : Scope  NumInputPorts=3
      settings: ActiveDisplayYMinimum=-2.2277455738782104  ActiveDisplayYMaximum=0.24752728598646778  DataLoggingVariableName=ScopeData3
  speed_reference_generator : Subsystem
  torque_reference : Subsystem
  udc_acquisition : Subsystem
  duvw : Outport  VectorParamsAs1DForOutWhenUnconnected=off
  local_time_corr : Outport  Port=2
  master_torque_ref : Outport  Port=3  VectorParamsAs1DForOutWhenUnconnected=off
  tag scope: isd_uvw_inv_mod1=scoped, local_time=scoped, omegad_pu_im=scoped, phased_im=scoped, udcd_pu_inv_mod1=scoped
  wires:
  speed_reference_generator/1(omega_ref_pu) -> Speed control/2(rotor speed ref), Bus Creator/2  "omega_ref_pu"
  Bus Creator/1 -> speed tracking/1  "speed_tracking"
  Variant Source/1 -> current_ctrl/1(torque_ref), speed tracking/2, master_torque_ref/1  "torque reference"
  [ux_pu_mod1] -> Mux2/1  "usx_ctrl"
  [uy_pu_mod1] -> Mux2/2  "usy_ctrl"
  Mux2/1 -> speed tracking/3
  [u_mot_pu_mod1] -> Mux2/3  "us_ctrl"
  omega_pu/2(omega_pu) -> Bus Creator/1, Speed control/1(rotor speed)  "omega_hat_pu"
  omega_pu/1(abs(omega_pu)) -> torque_reference/1(rotor speed)
  torque_reference/1(torque_ref) -> Variant Source/1  "iq_ref"
  Speed control/1(torque_ref) -> Variant Source/2  "iq_ref"
  udc_acquisition/1(udcd_pu) -> [udcd_pu_inv_mod1]
  udc_pu/1 -> udc_acquisition/1(udc_pu)
  is_uvw/1 -> is inv quantizzation and one step delay/1(is_abc_pu)
  is inv quantizzation and one step delay/1(isd_abc_pu) -> [isd_uvw_inv_mod1]
  local_time/1 -> To Workspace1/1, [local_time]
  current_ctrl/1(uab) -> space_vector/1(uab_out)
  space_vector/1(duvw) -> duvw/1
  master_time/1 -> phase_compensation_1/2(master_time)
  [local_time] -> phase_compensation_1/1(local_time)
  phase_compensation_1/1(y) -> local_time_corr/1
  phase_acquisition/1(phased_psm) -> [phased_im]
  rotor_phase_elec_im/1 -> phase_acquisition/1(phase_psm)
  rotor_speed_elec_im/1 -> phase_acquisition1/1(omega_psm)
  phase_acquisition1/1(omega_pu_psm) -> [omegad_pu_im]

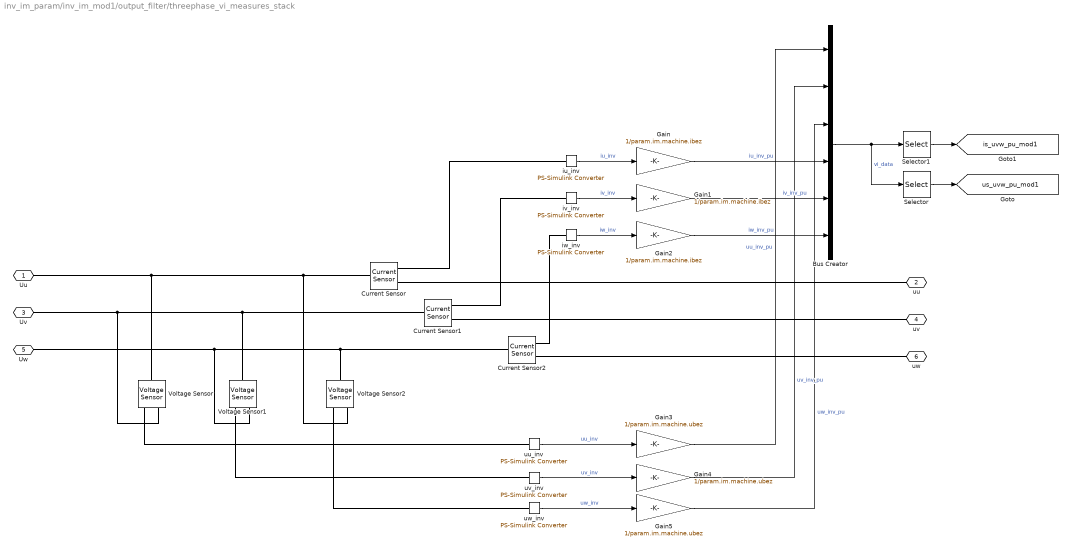
== system inv_im_param/inv_im_mod1/output_filter/threephase_vi_measures_stack ==
  Bus Creator : BusCreator  Inputs=6
  Current Sensor : fl_lib/Electrical/Electrical Sensors/Current Sensor
  Current Sensor1 : fl_lib/Electrical/Electrical Sensors/Current Sensor
  Current Sensor2 : fl_lib/Electrical/Electrical Sensors/Current Sensor
  Gain : Gain  Gain=1/param.im.machine.ibez
  Gain1 : Gain  Gain=1/param.im.machine.ibez
  Gain2 : Gain  Gain=1/param.im.machine.ibez
  Gain3 : Gain  Gain=1/param.im.machine.ubez
  Gain4 : Gain  Gain=1/param.im.machine.ubez
  Gain5 : Gain  Gain=1/param.im.machine.ubez
  Selector : Selector  InputPortWidth=6  IndexOptions=Index vector (dialog)  Indices=[1 2 3]  OutputSizes=1  RuntimeRangeChecks=off
  Selector1 : Selector  InputPortWidth=6  IndexOptions=Index vector (dialog)  Indices=[4 5 6]  OutputSizes=1  RuntimeRangeChecks=off
  Voltage Sensor : fl_lib/Electrical/Electrical Sensors/Voltage Sensor
  Voltage Sensor1 : fl_lib/Electrical/Electrical Sensors/Voltage Sensor
  Voltage Sensor2 : fl_lib/Electrical/Electrical Sensors/Voltage Sensor
  iu_inv : nesl_utility/PS-Simulink Converter  PhysicalDomain=network_engine_domain  SubClassName=ps_output  LeftPortType=input  RightPortType=output  PseudoPeriodic=off  Frequencies=[]  VectorFormat=1-D array  Unit=A  AffineConversion=off
  iv_inv : nesl_utility/PS-Simulink Converter  PhysicalDomain=network_engine_domain  SubClassName=ps_output  LeftPortType=input  RightPortType=output  PseudoPeriodic=off  Frequencies=[]  VectorFormat=1-D array  Unit=A  AffineConversion=off
  iw_inv : nesl_utility/PS-Simulink Converter  PhysicalDomain=network_engine_domain  SubClassName=ps_output  LeftPortType=input  RightPortType=output  PseudoPeriodic=off  Frequencies=[]  VectorFormat=1-D array  Unit=A  AffineConversion=off
  uu_inv : nesl_utility/PS-Simulink Converter  PhysicalDomain=network_engine_domain  SubClassName=ps_output  LeftPortType=input  RightPortType=output  PseudoPeriodic=off  Frequencies=[]  VectorFormat=1-D array  Unit=V  AffineConversion=off
  uv_inv : nesl_utility/PS-Simulink Converter  PhysicalDomain=network_engine_domain  SubClassName=ps_output  LeftPortType=input  RightPortType=output  PseudoPeriodic=off  Frequencies=[]  VectorFormat=1-D array  Unit=V  AffineConversion=off
  uw_inv : nesl_utility/PS-Simulink Converter  PhysicalDomain=network_engine_domain  SubClassName=ps_output  LeftPortType=input  RightPortType=output  PseudoPeriodic=off  Frequencies=[]  VectorFormat=1-D array  Unit=V  AffineConversion=off
  Uu : PMIOPort  Side=Left
  uu : PMIOPort  Port=2  Side=Right
  Uv : PMIOPort  Port=3  Side=Left
  uv : PMIOPort  Port=4  Side=Right
  Uw : PMIOPort  Port=5  Side=Left
  uw : PMIOPort  Port=6  Side=Right
  tag scope: is_uvw_pu_mod1=global, us_uvw_pu_mod1=global
  wires:
  Bus Creator/1 -> Selector/1, Selector1/1  "vi_data"
  Selector/1 -> [us_uvw_pu_mod1]
  iv_inv/1 -> Gain1/1  "iv_inv"
  iu_inv/1 -> Gain/1  "iu_inv"
  iw_inv/1 -> Gain2/1  "iw_inv"
  uu_inv/1 -> Gain3/1  "uu_inv"
  uv_inv/1 -> Gain4/1  "uv_inv"
  uw_inv/1 -> Gain5/1  "uw_inv"
  Selector1/1 -> [is_uvw_pu_mod1]
  Gain/1 -> Bus Creator/4  "iu_inv_pu"
  Gain1/1 -> Bus Creator/5  "iv_inv_pu"
  Gain2/1 -> Bus Creator/6  "iw_inv_pu"
  Gain3/1 -> Bus Creator/1  "uu_inv_pu"
  Gain4/1 -> Bus Creator/2  "uv_inv_pu"
  Gain5/1 -> Bus Creator/3  "uw_inv_pu"
  connections:
  Current Sensor1/LConn1 -- Voltage Sensor1/LConn1 -- Voltage Sensor/RConn2 -- Uv/RConn1
  Voltage Sensor/RConn1 -- uu_inv/LConn1
  Current Sensor/RConn2 -- uu/RConn1
  Voltage Sensor1/RConn1 -- uv_inv/LConn1
  Voltage Sensor2/LConn1 -- Current Sensor2/LConn1 -- Voltage Sensor1/RConn2 -- Uw/RConn1
  Current Sensor/LConn1 -- Voltage Sensor2/RConn2 -- Voltage Sensor/LConn1 -- Uu/RConn1
  Current Sensor1/RConn2 -- uv/RConn1
  Voltage Sensor2/RConn1 -- uw_inv/LConn1
  iv_inv/LConn1 -- Current Sensor1/RConn1
  iu_inv/LConn1 -- Current Sensor/RConn1
  iw_inv/LConn1 -- Current Sensor2/RConn1
  Current Sensor2/RConn2 -- uw/RConn1
